simulink library "Body_Utilities"  (R2025a)
settings: Solver=VariableStepAuto  StartTime=0.0  StopTime=10.0  RelTol=1e-3
undefined symbols (not defined in the file or in its folder): Init, Vehicle, X, Y, Z
libraries: nesl_utility x38, sm_lib x9
Description:
  | Simscape Vehicle Templates Library
  | 
  | Copyright 2018-2026 The MathWorks, Inc.
settings Model: Creator=smiller  LastModifiedBy=smiller
settings OptimizationCC: ReuseModelBlockBuffer=off
settings ModelReferenceCC: EnableRefExpFcnMdlSchedulingChecks=on
settings RTWCC: GPUComputeCapability=3.5

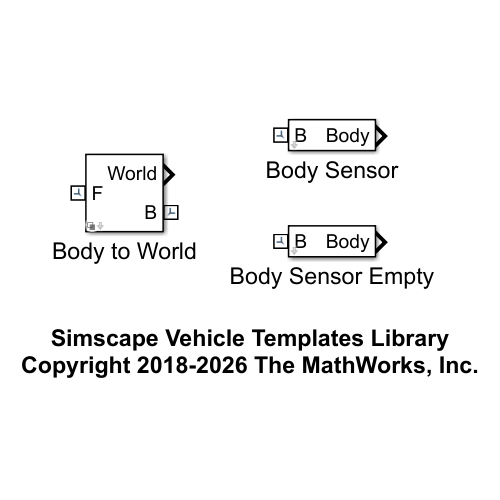
[thumbnail: Simulink's stored preview of the top-level diagram]
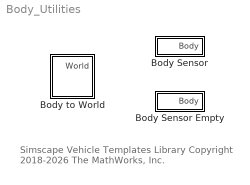
== system Body_Utilities ==
  note: Simscape Vehicle Templates Library
      | Copyright 2018-2026 The MathWorks, Inc.
  Body Sensor : Subsystem  mask{offset_body_sensor=Vehicle.Chassis.Body.sCG.Value}
      mask prompts: offset_body_sensor "Sensor Frame Offset [x y z] (m)"
  Body Sensor Empty : Subsystem  mask{offset_body_sensor=Vehicle.Chassis.Body.sCG.Value}
      mask prompts: offset_body_sensor "Sensor Frame Offset [x y z] (m)"
  Body to World : Subsystem  Variant=on  VariantControlMode=label  VariantControl=Choice  LabelModeActiveChoice=Free  mask{popup_BodyToWorld=Free, SpecifyPosTarget=on}
      mask prompts: popup_BodyToWorld "Body To World Connection"; SpecifyPosTarget "Specify Position Target"
      mask init:
      | bh = gcb;
      | b2w = get_param(bh,'popup_BodyToWorld');
      | set_param(bh,'LabelModeActiveChoice',b2w)
      | if(strcmp(b2w,'Free'))
      |     set_param([bh '/Free'],'SpecifyPosTarget',get_param(bh,'SpecifyPosTarget'));
      | end
      mask TypeOptions popup_BodyToWorld: Free | Rigid
      mask Display: disp(' ')

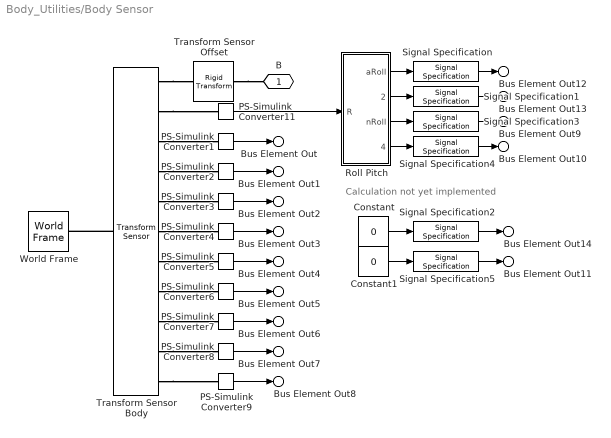
== system Body_Utilities/Body Sensor ==
  note: Calculation not yet implemented
  Constant : Constant  Value=0
  Constant1 : Constant  Value=0
  PS-Simulink Converter1 : nesl_utility/PS-Simulink Converter  PhysicalDomain=network_engine_domain  SubClassName=ps_output  LeftPortType=input  RightPortType=output  PseudoPeriodic=off  Frequencies=[]  VectorFormat=1-D array  Unit=m  AffineConversion=off
  PS-Simulink Converter11 : nesl_utility/PS-Simulink Converter  PhysicalDomain=network_engine_domain  SubClassName=ps_output  LeftPortType=input  RightPortType=output  PseudoPeriodic=off  Frequencies=[]  VectorFormat=1-D array  Unit=1  AffineConversion=off
  PS-Simulink Converter2 : nesl_utility/PS-Simulink Converter  PhysicalDomain=network_engine_domain  SubClassName=ps_output  LeftPortType=input  RightPortType=output  PseudoPeriodic=off  Frequencies=[]  VectorFormat=1-D array  Unit=m  AffineConversion=off
  PS-Simulink Converter3 : nesl_utility/PS-Simulink Converter  PhysicalDomain=network_engine_domain  SubClassName=ps_output  LeftPortType=input  RightPortType=output  PseudoPeriodic=off  Frequencies=[]  VectorFormat=1-D array  Unit=m  AffineConversion=off
  PS-Simulink Converter4 : nesl_utility/PS-Simulink Converter  PhysicalDomain=network_engine_domain  SubClassName=ps_output  LeftPortType=input  RightPortType=output  PseudoPeriodic=off  Frequencies=[]  VectorFormat=1-D array  Unit=m/s  AffineConversion=off
  PS-Simulink Converter5 : nesl_utility/PS-Simulink Converter  PhysicalDomain=network_engine_domain  SubClassName=ps_output  LeftPortType=input  RightPortType=output  PseudoPeriodic=off  Frequencies=[]  VectorFormat=1-D array  Unit=m/s  AffineConversion=off
  PS-Simulink Converter6 : nesl_utility/PS-Simulink Converter  PhysicalDomain=network_engine_domain  SubClassName=ps_output  LeftPortType=input  RightPortType=output  PseudoPeriodic=off  Frequencies=[]  VectorFormat=1-D array  Unit=m/s  AffineConversion=off
  PS-Simulink Converter7 : nesl_utility/PS-Simulink Converter  PhysicalDomain=network_engine_domain  SubClassName=ps_output  LeftPortType=input  RightPortType=output  PseudoPeriodic=off  Frequencies=[]  VectorFormat=1-D array  Unit=m/s^2  AffineConversion=off
  PS-Simulink Converter8 : nesl_utility/PS-Simulink Converter  PhysicalDomain=network_engine_domain  SubClassName=ps_output  LeftPortType=input  RightPortType=output  PseudoPeriodic=off  Frequencies=[]  VectorFormat=1-D array  Unit=m/s^2  AffineConversion=off
  PS-Simulink Converter9 : nesl_utility/PS-Simulink Converter  PhysicalDomain=network_engine_domain  SubClassName=ps_output  LeftPortType=input  RightPortType=output  PseudoPeriodic=off  Frequencies=[]  VectorFormat=1-D array  Unit=m/s^2  AffineConversion=off
  Roll Pitch : Subsystem
  Signal Specification : SignalSpecification  Unit=rad
  Signal Specification1 : SignalSpecification  Unit=rad
  Signal Specification2 : SignalSpecification  Unit=rad
  Signal Specification3 : SignalSpecification  Unit=rad/s
  Signal Specification4 : SignalSpecification  Unit=rad/s
  Signal Specification5 : SignalSpecification  Unit=rad/s
  Transform Sensor Offset : sm_lib/Frames and Transforms/Rigid Transform  RotationMethod=None  FollAlignAxisA=+X  BaseAlignAxisA=+Y  FollAlignAxisB=+Y  BaseAlignAxisB=+Z  RotationStandardAxis=+Z  RotationAngle=0.0  RotationAngleUnits=deg  RotationArbitraryAxis=[0 0 1]  RotationSequenceAxes=FollowerAxes  RotationSequence=XYX  RotationSequenceAngles=[0 0 0]  RotationSequenceAnglesUnits=deg  RotationMatrix=[1 0 0; 0 1 0; 0 0 1]  Quaternion=[1 0 0 0]  TranslationMethod=Cartesian  TranslationCartesianOffset=offset_body_sensor  TranslationCartesianOffsetUnits=m  TranslationStandardAxis=+Z  TranslationStandardOffset=0  TranslationStandardOffsetUnits=m  TranslationROffset=0  TranslationROffsetUnits=m  TranslationThetaOffset=0  TranslationThetaOffsetUnits=deg  TranslationZOffset=0  TranslationZOffsetUnits=m
  Transform Sensor Body : sm_lib/Frames and Transforms/Transform Sensor  MeasurementFrame=NonRotatingFollower  RotationSequence=XYX  SenseAngle=off  SenseAxis=off  SenseQ=off  SenseR=on  SenseRotationSequence=off  SenseOmegaX=off  SenseOmegaY=off  SenseOmegaZ=off  SenseOmega=off  SenseQDot=off  SenseRDot=off  SenseRotationSequenceDot=off  SenseAlphaX=off  SenseAlphaY=off  SenseAlphaZ=off  SenseAlpha=off  SenseQDDot=off  SenseRDDot=off  SenseX=on  SenseY=on  SenseZ=on  SenseXYZ=off  SenseRad=off  SenseAzim=off  SenseDist=off  SenseInc=off  SenseXDot=on  SenseYDot=on  SenseZDot=on  SenseXYZDot=off  SenseRadDot=off  SenseAzimDot=off  SenseDistDot=off  SenseIncDot=off  SenseXDDot=on  SenseYDDot=on  SenseZDDot=on  SenseXYZDDot=off  SenseRadDDot=off  SenseAzimDDot=off  SenseDistDDot=off  SenseIncDDot=off
  World Frame : sm_lib/Frames and Transforms/World Frame
  B : PMIOPort  Side=Left
  Bus Element Out : Outport  VectorParamsAs1DForOutWhenUnconnected=off  PortName=Body  Element=x
  Bus Element Out1 : Outport  VectorParamsAs1DForOutWhenUnconnected=off  PortName=Body  Element=y
  Bus Element Out2 : Outport  VectorParamsAs1DForOutWhenUnconnected=off  PortName=Body  Element=z
  Bus Element Out3 : Outport  VectorParamsAs1DForOutWhenUnconnected=off  PortName=Body  Element=vx
  Bus Element Out4 : Outport  VectorParamsAs1DForOutWhenUnconnected=off  PortName=Body  Element=vy
  Bus Element Out5 : Outport  VectorParamsAs1DForOutWhenUnconnected=off  PortName=Body  Element=vz
  Bus Element Out6 : Outport  VectorParamsAs1DForOutWhenUnconnected=off  PortName=Body  Element=gx
  Bus Element Out7 : Outport  VectorParamsAs1DForOutWhenUnconnected=off  PortName=Body  Element=gy
  Bus Element Out8 : Outport  VectorParamsAs1DForOutWhenUnconnected=off  PortName=Body  Element=gz
  Bus Element Out9 : Outport  VectorParamsAs1DForOutWhenUnconnected=off  PortName=Body  Element=nRoll
  Bus Element Out10 : Outport  VectorParamsAs1DForOutWhenUnconnected=off  PortName=Body  Element=nPitch
  Bus Element Out11 : Outport  VectorParamsAs1DForOutWhenUnconnected=off  PortName=Body  Element=nYaw
  Bus Element Out12 : Outport  VectorParamsAs1DForOutWhenUnconnected=off  PortName=Body  Element=aRoll
  Bus Element Out13 : Outport  VectorParamsAs1DForOutWhenUnconnected=off  PortName=Body  Element=aPitch
  Bus Element Out14 : Outport  VectorParamsAs1DForOutWhenUnconnected=off  PortName=Body  Element=aYaw
  wires:
  Roll Pitch/1(aRoll) -> Signal Specification/1
  Roll Pitch/2(aPitch) -> Signal Specification1/1
  Roll Pitch/4(nPitch) -> Signal Specification4/1
  Roll Pitch/3(nRoll) -> Signal Specification3/1
  Constant1/1 -> Signal Specification5/1
  Constant/1 -> Signal Specification2/1
  Signal Specification5/1 -> Bus Element Out11/1
  Signal Specification4/1 -> Bus Element Out10/1
  Signal Specification3/1 -> Bus Element Out9/1
  Signal Specification2/1 -> Bus Element Out14/1
  Signal Specification1/1 -> Bus Element Out13/1
  Signal Specification/1 -> Bus Element Out12/1
  PS-Simulink Converter4/1 -> Bus Element Out3/1
  PS-Simulink Converter1/1 -> Bus Element Out/1
  PS-Simulink Converter3/1 -> Bus Element Out2/1
  PS-Simulink Converter5/1 -> Bus Element Out4/1
  PS-Simulink Converter8/1 -> Bus Element Out7/1
  PS-Simulink Converter2/1 -> Bus Element Out1/1
  PS-Simulink Converter7/1 -> Bus Element Out6/1
  PS-Simulink Converter6/1 -> Bus Element Out5/1
  PS-Simulink Converter11/1 -> Roll Pitch/1(R)
  PS-Simulink Converter9/1 -> Bus Element Out8/1
  connections:
  Transform Sensor Body/RConn1 -- Transform Sensor Offset/RConn1
  Transform Sensor Body/RConn6 -- PS-Simulink Converter4/LConn1
  Transform Sensor Body/RConn8 -- PS-Simulink Converter6/LConn1
  Transform Sensor Body/RConn9 -- PS-Simulink Converter7/LConn1
  Transform Sensor Body/RConn10 -- PS-Simulink Converter8/LConn1
  Transform Sensor Offset/LConn1 -- B/RConn1
  Transform Sensor Body/LConn1 -- World Frame/RConn1
  Transform Sensor Body/RConn3 -- PS-Simulink Converter1/LConn1
  Transform Sensor Body/RConn7 -- PS-Simulink Converter5/LConn1
  Transform Sensor Body/RConn2 -- PS-Simulink Converter11/LConn1
  Transform Sensor Body/RConn11 -- PS-Simulink Converter9/LConn1
  Transform Sensor Body/RConn4 -- PS-Simulink Converter2/LConn1
  Transform Sensor Body/RConn5 -- PS-Simulink Converter3/LConn1

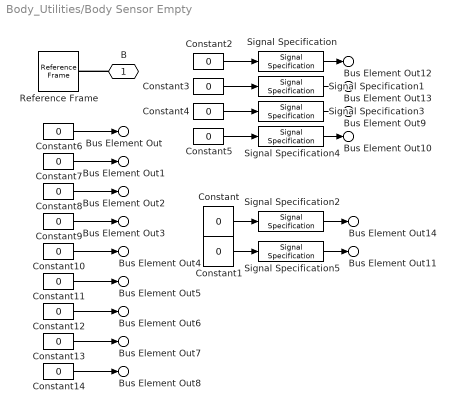
== system Body_Utilities/Body Sensor Empty ==
  Constant{,1..14} (15 alike) : Constant  Value=0
  Reference Frame : sm_lib/Frames and Transforms/Reference Frame
  Signal Specification : SignalSpecification  Unit=rad
  Signal Specification1 : SignalSpecification  Unit=rad
  Signal Specification2 : SignalSpecification  Unit=rad
  Signal Specification3 : SignalSpecification  Unit=rad/s
  Signal Specification4 : SignalSpecification  Unit=rad/s
  Signal Specification5 : SignalSpecification  Unit=rad/s
  B : PMIOPort  Side=Left
  Bus Element Out : Outport  VectorParamsAs1DForOutWhenUnconnected=off  PortName=Body  Element=x
  Bus Element Out1 : Outport  VectorParamsAs1DForOutWhenUnconnected=off  PortName=Body  Element=y
  Bus Element Out2 : Outport  VectorParamsAs1DForOutWhenUnconnected=off  PortName=Body  Element=z
  Bus Element Out3 : Outport  VectorParamsAs1DForOutWhenUnconnected=off  PortName=Body  Element=vx
  Bus Element Out4 : Outport  VectorParamsAs1DForOutWhenUnconnected=off  PortName=Body  Element=vy
  Bus Element Out5 : Outport  VectorParamsAs1DForOutWhenUnconnected=off  PortName=Body  Element=vz
  Bus Element Out6 : Outport  VectorParamsAs1DForOutWhenUnconnected=off  PortName=Body  Element=gx
  Bus Element Out7 : Outport  VectorParamsAs1DForOutWhenUnconnected=off  PortName=Body  Element=gy
  Bus Element Out8 : Outport  VectorParamsAs1DForOutWhenUnconnected=off  PortName=Body  Element=gz
  Bus Element Out9 : Outport  VectorParamsAs1DForOutWhenUnconnected=off  PortName=Body  Element=nRoll
  Bus Element Out10 : Outport  VectorParamsAs1DForOutWhenUnconnected=off  PortName=Body  Element=nPitch
  Bus Element Out11 : Outport  VectorParamsAs1DForOutWhenUnconnected=off  PortName=Body  Element=nYaw
  Bus Element Out12 : Outport  VectorParamsAs1DForOutWhenUnconnected=off  PortName=Body  Element=aRoll
  Bus Element Out13 : Outport  VectorParamsAs1DForOutWhenUnconnected=off  PortName=Body  Element=aPitch
  Bus Element Out14 : Outport  VectorParamsAs1DForOutWhenUnconnected=off  PortName=Body  Element=aYaw
  wires:
  Constant14/1 -> Bus Element Out8/1
  Constant11/1 -> Bus Element Out5/1
  Constant12/1 -> Bus Element Out6/1
  Constant7/1 -> Bus Element Out1/1
  Constant13/1 -> Bus Element Out7/1
  Constant10/1 -> Bus Element Out4/1
  Constant8/1 -> Bus Element Out2/1
  Constant6/1 -> Bus Element Out/1
  Constant9/1 -> Bus Element Out3/1
  Signal Specification/1 -> Bus Element Out12/1
  Signal Specification1/1 -> Bus Element Out13/1
  Signal Specification2/1 -> Bus Element Out14/1
  Signal Specification3/1 -> Bus Element Out9/1
  Signal Specification4/1 -> Bus Element Out10/1
  Signal Specification5/1 -> Bus Element Out11/1
  Constant/1 -> Signal Specification2/1
  Constant1/1 -> Signal Specification5/1
  Constant4/1 -> Signal Specification3/1
  Constant5/1 -> Signal Specification4/1
  Constant3/1 -> Signal Specification1/1
  Constant2/1 -> Signal Specification/1
  connections:
  B/RConn1 -- Reference Frame/RConn1

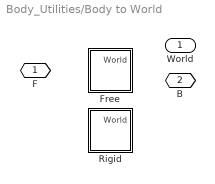
== system Body_Utilities/Body to World ==
  Free : Subsystem  VariantControl=Free  mask(Body to World){Init=Init.Chassis, SpecifyPosTarget=on}
      mask prompts: Init "Initial Values"; SpecifyPosTarget "Specify Position Target"
      mask help: Models the connection between the vehicle body and world. Permits 6 degrees of freedom and sets the initial position, orientation, and speed of the vehicle body.
      mask init:
      | initial_aveh = [Init.aChassis.Value(3) Init.aChassis.Value(2) Init.aChassis.Value(1)];
      | rotmat_ypr = sm_car_yawpitchroll_to_rotmat(Init.aChassis.Value(3),Init.aChassis.Value(2),Init.aChassis.Value(1));
      | initial_vveh = rotmat_ypr*(Init.vChassis.Value)';
      | 
      | sptState = get_param(gcb,'SpecifyPosTarget');
      | 
      | set_param([gcb '/Body World Joint'],...
      |         'PxPositionTargetSpecify',sptState,...
      |         'PyPositionTargetSpecify',sptState,...
      |         'PzPositionTargetSpecify',sptState,...
      |         'SphPositionTargetSpecify',sptState,...
      |         'PxVelocityTargetSpecify',sptState,...
      |         'PyVelocityTargetSpecify',sptState,...
      |         'PzVelocityTargetSpecify',sptState,...
      |         'SphVelocityTargetSpecify',sptState...
      |         );
      mask Help: web('sm_car_doc_body_to_world.html')
  Rigid : Subsystem  VariantControl=Rigid  mask(Body to World){Init=Init.Chassis}
      mask prompts: Init "Initial Values"
      mask help: Models the connection between the vehicle body and world. Permits 6 degrees of freedom and sets the initial position, orientation, and speed of the vehicle body.
      mask init:
      | initial_aveh = [Init.aChassis.Value(3) Init.aChassis.Value(2) Init.aChassis.Value(1)];
      | rotmat_ypr = sm_car_yawpitchroll_to_rotmat(Init.aChassis.Value(3),Init.aChassis.Value(2),Init.aChassis.Value(1));
      | initial_vveh = rotmat_ypr*(Init.vChassis.Value)';
      mask Help: web('sm_car_doc_body_to_world.html')
  F : PMIOPort  Side=Left
  B : PMIOPort  Port=2  Side=Right
  World : Outport

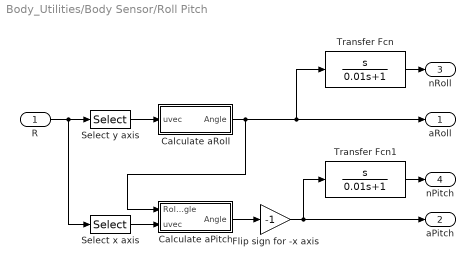
== system Body_Utilities/Body Sensor/Roll Pitch ==
  R : Inport
  Calculate aPitch : Subsystem
  Calculate aRoll : Subsystem
  "Flip sign for -x axis " : Gain  Gain=-1
  Select x axis : Selector  NumberOfDimensions=2  InputPortWidth=2  IndexOptions=Index vector (dialog),Index vector (dialog)  Indices=[1 2 3],1  OutputSizes=1,1
  Select y axis : Selector  NumberOfDimensions=2  InputPortWidth=2  IndexOptions=Index vector (dialog),Index vector (dialog)  Indices=[1 2 3],2  OutputSizes=1,1
  Transfer Fcn : TransferFcn  Numerator=[1 0]  Denominator=[0.01 1]
  Transfer Fcn1 : TransferFcn  Numerator=[1 0]  Denominator=[0.01 1]
  aRoll : Outport  VectorParamsAs1DForOutWhenUnconnected=off
  aPitch : Outport  Port=2  VectorParamsAs1DForOutWhenUnconnected=off
  nRoll : Outport  Port=3  VectorParamsAs1DForOutWhenUnconnected=off
  nPitch : Outport  Port=4  VectorParamsAs1DForOutWhenUnconnected=off
  wires:
  Transfer Fcn1/1 -> nPitch/1
  Transfer Fcn/1 -> nRoll/1
  Calculate aRoll/1(Angle) -> Calculate aPitch/1(Roll Angle), aRoll/1, Transfer Fcn/1
  "Flip sign for -x axis "/1 -> Transfer Fcn1/1, aPitch/1
  Select y axis/1 -> Calculate aRoll/1(uvec)
  R/1 -> Select x axis/1, Select y axis/1
  Select x axis/1 -> Calculate aPitch/2(uvec)
  Calculate aPitch/1(Angle) -> "Flip sign for -x axis "/1

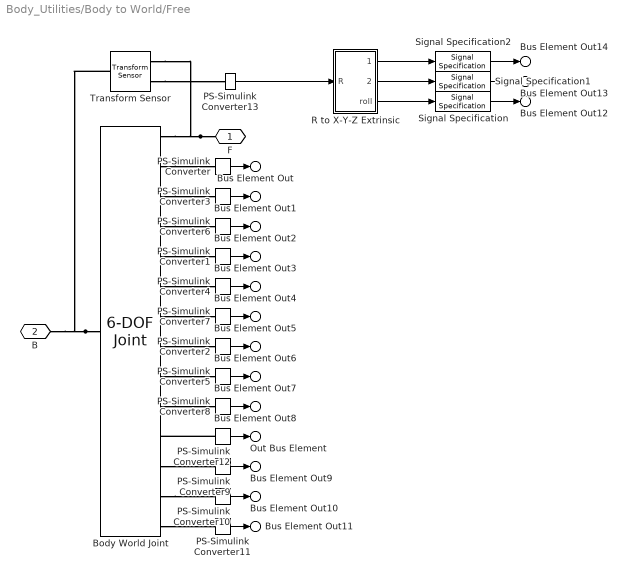
== system Body_Utilities/Body to World/Free ==
  Body World Joint : sm_lib/Joints/6-DOF Joint  JointMode=Normal  CompositeWrenchDir=FollowerOnBase  CompositeWrenchFrame=BaseFrame  SenseConstraintForce=off  SenseConstraintTorque=off  SenseTotalForce=off  SenseTotalTorque=off  PxPositionTargetSpecify=on  PxPositionTargetPriority=Low  PxPositionTargetValue=Init.sChassis.Value(1)  PxPositionTargetValueUnits=m  PxVelocityTargetSpecify=on  PxVelocityTargetPriority=Low  PxVelocityTargetValue=initial_vveh(1)  PxVelocityTargetValueUnits=m/s  PxEquilibriumPosition=0  PxEquilibriumPositionUnits=m  PxSpringStiffness=0  PxSpringStiffnessUnits=N/m  PxDampingCoefficient=0  PxDampingCoefficientUnits=N/(m/s)  PxLowerLimitSpecify=off  PxLowerLimitBound=-1  PxLowerLimitBoundUnits=m  PxLowerLimitStiffness=1e6  PxLowerLimitStiffnessUnits=N/m  PxLowerLimitDamping=1e3  PxLowerLimitDampingUnits=N/(m/s)  PxLowerLimitTransitionRegionWidth=1e-4  PxLowerLimitTransitionRegionWidthUnits=m  PxUpperLimitSpecify=off  PxUpperLimitBound=1  PxUpperLimitBoundUnits=m  PxUpperLimitStiffness=1e6  PxUpperLimitStiffnessUnits=N/m  PxUpperLimitDamping=1e3  PxUpperLimitDampingUnits=N/(m/s)  PxUpperLimitTransitionRegionWidth=1e-4  PxUpperLimitTransitionRegionWidthUnits=m  PxTorqueActuationMode=NoTorque  PxMotionActuationMode=ComputedMotion  PxSensePosition=on  PxSenseVelocity=on  PxSenseAcceleration=on  PxSenseTorqueForce=off  PxSenseLowerLimitTorqueForce=off  PxSenseUpperLimitTorqueForce=off  PyPositionTargetSpecify=on  PyPositionTargetPriority=Low  PyPositionTargetValue=Init.sChassis.Value(2)  PyPositionTargetValueUnits=m  PyVelocityTargetSpecify=on  PyVelocityTargetPriority=Low  PyVelocityTargetValue=initial_vveh(2)  PyVelocityTargetValueUnits=m/s  PyEquilibriumPosition=0  PyEquilibriumPositionUnits=m  PySpringStiffness=0  PySpringStiffnessUnits=N/m  PyDampingCoefficient=0  PyDampingCoefficientUnits=N/(m/s)  PyLowerLimitSpecify=off  PyLowerLimitBound=-1  PyLowerLimitBoundUnits=m  PyLowerLimitStiffness=1e6  PyLowerLimitStiffnessUnits=N/m  PyLowerLimitDamping=1e3  PyLowerLimitDampingUnits=N/(m/s)  PyLowerLimitTransitionRegionWidth=1e-4  PyLowerLimitTransitionRegionWidthUnits=m  PyUpperLimitSpecify=off  PyUpperLimitBound=1  PyUpperLimitBoundUnits=m  PyUpperLimitStiffness=1e6  PyUpperLimitStiffnessUnits=N/m  PyUpperLimitDamping=1e3  PyUpperLimitDampingUnits=N/(m/s)  PyUpperLimitTransitionRegionWidth=1e-4  PyUpperLimitTransitionRegionWidthUnits=m  PyTorqueActuationMode=NoTorque  PyMotionActuationMode=ComputedMotion  PySensePosition=on  PySenseVelocity=on  PySenseAcceleration=on  PySenseTorqueForce=off  PySenseLowerLimitTorqueForce=off  PySenseUpperLimitTorqueForce=off  PzPositionTargetSpecify=on  PzPositionTargetPriority=Low  PzPositionTargetValue=Init.sChassis.Value(3)  PzPositionTargetValueUnits=m  PzVelocityTargetSpecify=on  PzVelocityTargetPriority=Low  PzVelocityTargetValue=initial_vveh(3)  PzVelocityTargetValueUnits=m/s  PzEquilibriumPosition=0  PzEquilibriumPositionUnits=m  PzSpringStiffness=0  PzSpringStiffnessUnits=N/m  PzDampingCoefficient=0  PzDampingCoefficientUnits=N/(m/s)  PzLowerLimitSpecify=off  PzLowerLimitBound=-1  PzLowerLimitBoundUnits=m  PzLowerLimitStiffness=1e6  PzLowerLimitStiffnessUnits=N/m  PzLowerLimitDamping=1e3  PzLowerLimitDampingUnits=N/(m/s)  PzLowerLimitTransitionRegionWidth=1e-4  PzLowerLimitTransitionRegionWidthUnits=m  PzUpperLimitSpecify=off  PzUpperLimitBound=1  PzUpperLimitBoundUnits=m  PzUpperLimitStiffness=1e6  PzUpperLimitStiffnessUnits=N/m  PzUpperLimitDamping=1e3  PzUpperLimitDampingUnits=N/(m/s)  PzUpperLimitTransitionRegionWidth=1e-4  PzUpperLimitTransitionRegionWidthUnits=m  PzTorqueActuationMode=NoTorque  PzMotionActuationMode=ComputedMotion  PzSensePosition=on  PzSenseVelocity=on  PzSenseAcceleration=on  PzSenseTorqueForce=off  PzSenseLowerLimitTorqueForce=off  PzSenseUpperLimitTorqueForce=off  SphPositionTargetSpecify=on  SphPositionTargetPriority=Low  SphPositionTargetRotationMethod=RotationSequence  SphPositionTargetFollAlignAxisA=+X  SphPositionTargetBaseAlignAxisA=+Y  SphPositionTargetFollAlignAxisB=+Y  SphPositionTargetBaseAlignAxisB=+Z  SphPositionTargetRotationStandardAxis=+Z  SphPositionTargetRotationAngle=0.0  SphPositionTargetRotationAngleUnits=deg  SphPositionTargetRotationArbitraryAxis=[0 0 1]  SphPositionTargetRotationSequenceAxes=FollowerAxes  SphPositionTargetRotationSequence=ZYX  SphPositionTargetRotationSequenceAngles=initial_aveh  SphPositionTargetRotationSequenceAnglesUnits=rad  SphPositionTargetRotationMatrix=[1 0 0; 0 1 0; 0 0 1]  SphPositionTargetQuaternion=[1 0 0 0]  SphVelocityTargetSpecify=on  SphVelocityTargetPriority=Low  SphVelocityTargetValue=[0 0 0]  SphVelocityTargetValueUnits=deg/s  SphVelocityTargetInFollowerFrame=on  SphEqPosRotationMethod=None  SphEqPosFollAlignAxisA=+X  SphEqPosBaseAlignAxisA=+Y  SphEqPosFollAlignAxisB=+Y  SphEqPosBaseAlignAxisB=+Z  SphEqPosRotationStandardAxis=+Z  SphEqPosRotationAngle=0.0  SphEqPosRotationAngleUnits=deg  SphEqPosRotationArbitraryAxis=[0 0 1]  SphEqPosRotationSequenceAxes=FollowerAxes  SphEqPosRotationSequence=XYX  SphEqPosRotationSequenceAngles=[0 0 0]  SphEqPosRotationSequenceAnglesUnits=deg  SphEqPosRotationMatrix=[1 0 0; 0 1 0; 0 0 1]  SphEqPosQuaternion=[1 0 0 0]  SphSpringStiffness=0  SphSpringStiffnessUnits=N*m/deg  SphDampingCoefficient=0  SphDampingCoefficientUnits=N*m/(deg/s)  SphLowerLimitSpecify=off  SphLowerLimitBound=15  SphLowerLimitBoundUnits=deg  SphLowerLimitStiffness=1e4  SphLowerLimitStiffnessUnits=N*m/deg  SphLowerLimitDamping=10  SphLowerLimitDampingUnits=N*m/(deg/s)  SphLowerLimitTransitionRegionWidth=0.1  SphLowerLimitTransitionRegionWidthUnits=deg  SphUpperLimitSpecify=off  SphUpperLimitBound=45  SphUpperLimitBoundUnits=deg  SphUpperLimitStiffness=1e4  SphUpperLimitStiffnessUnits=N*m/deg  SphUpperLimitDamping=10  SphUpperLimitDampingUnits=N*m/(deg/s)  SphUpperLimitTransitionRegionWidth=0.1  SphUpperLimitTransitionRegionWidthUnits=deg  SphTorqueActuationMode=NoTorque  SphActuateTorqueX=off  SphActuateTorqueY=off  SphActuateTorqueZ=off  SphActuateTorque=off  SphActuationFrame=BaseFrame  SphSensePosition=on  SphSenseVelocityX=on  SphSenseVelocityY=on  SphSenseVelocityZ=on  SphSenseVelocity=off  SphSenseAccelerationX=off  SphSenseAccelerationY=off  SphSenseAccelerationZ=off  SphSenseAcceleration=off  SphSenseLowerLimitTorqueMag=off  SphSenseUpperLimitTorqueMag=off  SphSensingFrame=BaseFrame
  PS-Simulink Converter : nesl_utility/PS-Simulink Converter  PhysicalDomain=network_engine_domain  SubClassName=ps_output  LeftPortType=input  RightPortType=output  PseudoPeriodic=off  Frequencies=[]  VectorFormat=1-D array  Unit=m  AffineConversion=off
  PS-Simulink Converter1 : nesl_utility/PS-Simulink Converter  PhysicalDomain=network_engine_domain  SubClassName=ps_output  LeftPortType=input  RightPortType=output  PseudoPeriodic=off  Frequencies=[]  VectorFormat=1-D array  Unit=m  AffineConversion=off
  PS-Simulink Converter10 : nesl_utility/PS-Simulink Converter  PhysicalDomain=network_engine_domain  SubClassName=ps_output  LeftPortType=input  RightPortType=output  PseudoPeriodic=off  Frequencies=[]  VectorFormat=1-D array  Unit=rad/s  AffineConversion=off
  PS-Simulink Converter11 : nesl_utility/PS-Simulink Converter  PhysicalDomain=network_engine_domain  SubClassName=ps_output  LeftPortType=input  RightPortType=output  PseudoPeriodic=off  Frequencies=[]  VectorFormat=1-D array  Unit=rad/s  AffineConversion=off
  PS-Simulink Converter12 : nesl_utility/PS-Simulink Converter  PhysicalDomain=network_engine_domain  SubClassName=ps_output  LeftPortType=input  RightPortType=output  PseudoPeriodic=off  Frequencies=[]  VectorFormat=1-D array  Unit=1  AffineConversion=off
  PS-Simulink Converter13 : nesl_utility/PS-Simulink Converter  PhysicalDomain=network_engine_domain  SubClassName=ps_output  LeftPortType=input  RightPortType=output  PseudoPeriodic=off  Frequencies=[]  VectorFormat=1-D array  Unit=1  AffineConversion=off
  PS-Simulink Converter2 : nesl_utility/PS-Simulink Converter  PhysicalDomain=network_engine_domain  SubClassName=ps_output  LeftPortType=input  RightPortType=output  PseudoPeriodic=off  Frequencies=[]  VectorFormat=1-D array  Unit=m  AffineConversion=off
  PS-Simulink Converter3 : nesl_utility/PS-Simulink Converter  PhysicalDomain=network_engine_domain  SubClassName=ps_output  LeftPortType=input  RightPortType=output  PseudoPeriodic=off  Frequencies=[]  VectorFormat=1-D array  Unit=m/s  AffineConversion=off
  PS-Simulink Converter4 : nesl_utility/PS-Simulink Converter  PhysicalDomain=network_engine_domain  SubClassName=ps_output  LeftPortType=input  RightPortType=output  PseudoPeriodic=off  Frequencies=[]  VectorFormat=1-D array  Unit=m/s  AffineConversion=off
  PS-Simulink Converter5 : nesl_utility/PS-Simulink Converter  PhysicalDomain=network_engine_domain  SubClassName=ps_output  LeftPortType=input  RightPortType=output  PseudoPeriodic=off  Frequencies=[]  VectorFormat=1-D array  Unit=m/s  AffineConversion=off
  PS-Simulink Converter6 : nesl_utility/PS-Simulink Converter  PhysicalDomain=network_engine_domain  SubClassName=ps_output  LeftPortType=input  RightPortType=output  PseudoPeriodic=off  Frequencies=[]  VectorFormat=1-D array  Unit=m/s^2  AffineConversion=off
  PS-Simulink Converter7 : nesl_utility/PS-Simulink Converter  PhysicalDomain=network_engine_domain  SubClassName=ps_output  LeftPortType=input  RightPortType=output  PseudoPeriodic=off  Frequencies=[]  VectorFormat=1-D array  Unit=m/s^2  AffineConversion=off
  PS-Simulink Converter8 : nesl_utility/PS-Simulink Converter  PhysicalDomain=network_engine_domain  SubClassName=ps_output  LeftPortType=input  RightPortType=output  PseudoPeriodic=off  Frequencies=[]  VectorFormat=1-D array  Unit=m/s^2  AffineConversion=off
  PS-Simulink Converter9 : nesl_utility/PS-Simulink Converter  PhysicalDomain=network_engine_domain  SubClassName=ps_output  LeftPortType=input  RightPortType=output  PseudoPeriodic=off  Frequencies=[]  VectorFormat=1-D array  Unit=rad/s  AffineConversion=off
  R to X-Y-Z Extrinsic : Subsystem  mask(Rotation Matrix to X-Y-Z Extrinsic){}
      mask help: Computes roll / pitch / yaw values assuming they correspond to X, Y, and Z rotations, applied in that order and using extrinsic rotations (rotations applied about the fixed axes of the base frame). Does not handle case where Y (pitch) rotation is +/-90 degrees.
  Signal Specification : SignalSpecification  Unit=rad
  Signal Specification1 : SignalSpecification  Unit=rad
  Signal Specification2 : SignalSpecification  Unit=rad
  Transform Sensor : sm_lib/Frames and Transforms/Transform Sensor  MeasurementFrame=World  RotationSequence=XYX  SenseAngle=off  SenseAxis=off  SenseQ=off  SenseR=on  SenseRotationSequence=off  SenseOmegaX=off  SenseOmegaY=off  SenseOmegaZ=off  SenseOmega=off  SenseQDot=off  SenseRDot=off  SenseRotationSequenceDot=off  SenseAlphaX=off  SenseAlphaY=off  SenseAlphaZ=off  SenseAlpha=off  SenseQDDot=off  SenseRDDot=off  SenseX=off  SenseY=off  SenseZ=off  SenseXYZ=off  SenseRad=off  SenseAzim=off  SenseDist=off  SenseInc=off  SenseXDot=off  SenseYDot=off  SenseZDot=off  SenseXYZDot=off  SenseRadDot=off  SenseAzimDot=off  SenseDistDot=off  SenseIncDot=off  SenseXDDot=off  SenseYDDot=off  SenseZDDot=off  SenseXYZDDot=off  SenseRadDDot=off  SenseAzimDDot=off  SenseDistDDot=off  SenseIncDDot=off
  F : PMIOPort  Side=Left
  B : PMIOPort  Port=2  Side=Right
  Bus Element Out : Outport  VectorParamsAs1DForOutWhenUnconnected=off  PortName=World  Element=x
  Bus Element Out3 : Outport  VectorParamsAs1DForOutWhenUnconnected=off  PortName=World  Element=y
  Bus Element Out6 : Outport  VectorParamsAs1DForOutWhenUnconnected=off  PortName=World  Element=z
  Bus Element Out1 : Outport  VectorParamsAs1DForOutWhenUnconnected=off  PortName=World  Element=vx
  Bus Element Out4 : Outport  VectorParamsAs1DForOutWhenUnconnected=off  PortName=World  Element=vy
  Bus Element Out7 : Outport  VectorParamsAs1DForOutWhenUnconnected=off  PortName=World  Element=vz
  Bus Element Out2 : Outport  VectorParamsAs1DForOutWhenUnconnected=off  PortName=World  Element=gx
  Bus Element Out5 : Outport  VectorParamsAs1DForOutWhenUnconnected=off  PortName=World  Element=gy
  Bus Element Out8 : Outport  VectorParamsAs1DForOutWhenUnconnected=off  PortName=World  Element=gz
  Bus Element Out9 : Outport  VectorParamsAs1DForOutWhenUnconnected=off  PortName=World  Element=nRoll
  Bus Element Out10 : Outport  VectorParamsAs1DForOutWhenUnconnected=off  PortName=World  Element=nPitch
  Bus Element Out11 : Outport  VectorParamsAs1DForOutWhenUnconnected=off  PortName=World  Element=nYaw
  Bus Element Out12 : Outport  VectorParamsAs1DForOutWhenUnconnected=off  PortName=World  Element=aRoll
  Bus Element Out13 : Outport  VectorParamsAs1DForOutWhenUnconnected=off  PortName=World  Element=aPitch
  Bus Element Out14 : Outport  VectorParamsAs1DForOutWhenUnconnected=off  PortName=World  Element=aYaw
  Out Bus Element : Outport  VectorParamsAs1DForOutWhenUnconnected=off  PortName=World  Element=Q
  wires:
  R to X-Y-Z Extrinsic/1(yaw) -> Signal Specification2/1
  R to X-Y-Z Extrinsic/3(roll) -> Signal Specification/1
  R to X-Y-Z Extrinsic/2(pitch) -> Signal Specification1/1
  PS-Simulink Converter13/1 -> R to X-Y-Z Extrinsic/1(R)
  PS-Simulink Converter12/1 -> Out Bus Element/1
  PS-Simulink Converter11/1 -> Bus Element Out11/1
  PS-Simulink Converter10/1 -> Bus Element Out10/1
  Signal Specification/1 -> Bus Element Out12/1
  Signal Specification1/1 -> Bus Element Out13/1
  Signal Specification2/1 -> Bus Element Out14/1
  PS-Simulink Converter3/1 -> Bus Element Out1/1
  PS-Simulink Converter2/1 -> Bus Element Out6/1
  PS-Simulink Converter6/1 -> Bus Element Out2/1
  PS-Simulink Converter4/1 -> Bus Element Out4/1
  PS-Simulink Converter/1 -> Bus Element Out/1
  PS-Simulink Converter5/1 -> Bus Element Out7/1
  PS-Simulink Converter9/1 -> Bus Element Out9/1
  PS-Simulink Converter8/1 -> Bus Element Out8/1
  PS-Simulink Converter7/1 -> Bus Element Out5/1
  PS-Simulink Converter1/1 -> Bus Element Out3/1
  connections:
  Transform Sensor/RConn2 -- PS-Simulink Converter13/LConn1
  PS-Simulink Converter12/LConn1 -- Body World Joint/RConn11
  Body World Joint/RConn8 -- PS-Simulink Converter2/LConn1
  Body World Joint/RConn9 -- PS-Simulink Converter5/LConn1
  F/RConn1 -- Transform Sensor/RConn1 -- Body World Joint/RConn1
  Body World Joint/RConn3 -- PS-Simulink Converter3/LConn1
  Body World Joint/RConn10 -- PS-Simulink Converter8/LConn1
  Body World Joint/RConn4 -- PS-Simulink Converter6/LConn1
  Body World Joint/RConn2 -- PS-Simulink Converter/LConn1
  Body World Joint/RConn7 -- PS-Simulink Converter7/LConn1
  Body World Joint/RConn13 -- PS-Simulink Converter10/LConn1
  Body World Joint/RConn14 -- PS-Simulink Converter11/LConn1
  Body World Joint/RConn5 -- PS-Simulink Converter1/LConn1
  Body World Joint/LConn1 -- Transform Sensor/LConn1 -- B/RConn1
  Body World Joint/RConn12 -- PS-Simulink Converter9/LConn1
  Body World Joint/RConn6 -- PS-Simulink Converter4/LConn1

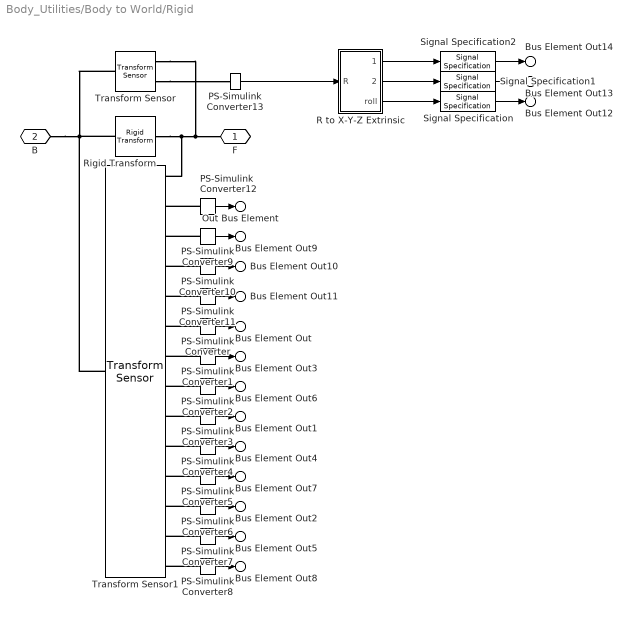
== system Body_Utilities/Body to World/Rigid ==
  PS-Simulink Converter : nesl_utility/PS-Simulink Converter  PhysicalDomain=network_engine_domain  SubClassName=ps_output  LeftPortType=input  RightPortType=output  PseudoPeriodic=off  Frequencies=[]  VectorFormat=1-D array  Unit=m  AffineConversion=off
  PS-Simulink Converter1 : nesl_utility/PS-Simulink Converter  PhysicalDomain=network_engine_domain  SubClassName=ps_output  LeftPortType=input  RightPortType=output  PseudoPeriodic=off  Frequencies=[]  VectorFormat=1-D array  Unit=m  AffineConversion=off
  PS-Simulink Converter10 : nesl_utility/PS-Simulink Converter  PhysicalDomain=network_engine_domain  SubClassName=ps_output  LeftPortType=input  RightPortType=output  PseudoPeriodic=off  Frequencies=[]  VectorFormat=1-D array  Unit=rad/s  AffineConversion=off
  PS-Simulink Converter11 : nesl_utility/PS-Simulink Converter  PhysicalDomain=network_engine_domain  SubClassName=ps_output  LeftPortType=input  RightPortType=output  PseudoPeriodic=off  Frequencies=[]  VectorFormat=1-D array  Unit=rad/s  AffineConversion=off
  PS-Simulink Converter12 : nesl_utility/PS-Simulink Converter  PhysicalDomain=network_engine_domain  SubClassName=ps_output  LeftPortType=input  RightPortType=output  PseudoPeriodic=off  Frequencies=[]  VectorFormat=1-D array  Unit=1  AffineConversion=off
  PS-Simulink Converter13 : nesl_utility/PS-Simulink Converter  PhysicalDomain=network_engine_domain  SubClassName=ps_output  LeftPortType=input  RightPortType=output  PseudoPeriodic=off  Frequencies=[]  VectorFormat=1-D array  Unit=1  AffineConversion=off
  PS-Simulink Converter2 : nesl_utility/PS-Simulink Converter  PhysicalDomain=network_engine_domain  SubClassName=ps_output  LeftPortType=input  RightPortType=output  PseudoPeriodic=off  Frequencies=[]  VectorFormat=1-D array  Unit=m  AffineConversion=off
  PS-Simulink Converter3 : nesl_utility/PS-Simulink Converter  PhysicalDomain=network_engine_domain  SubClassName=ps_output  LeftPortType=input  RightPortType=output  PseudoPeriodic=off  Frequencies=[]  VectorFormat=1-D array  Unit=m/s  AffineConversion=off
  PS-Simulink Converter4 : nesl_utility/PS-Simulink Converter  PhysicalDomain=network_engine_domain  SubClassName=ps_output  LeftPortType=input  RightPortType=output  PseudoPeriodic=off  Frequencies=[]  VectorFormat=1-D array  Unit=m/s  AffineConversion=off
  PS-Simulink Converter5 : nesl_utility/PS-Simulink Converter  PhysicalDomain=network_engine_domain  SubClassName=ps_output  LeftPortType=input  RightPortType=output  PseudoPeriodic=off  Frequencies=[]  VectorFormat=1-D array  Unit=m/s  AffineConversion=off
  PS-Simulink Converter6 : nesl_utility/PS-Simulink Converter  PhysicalDomain=network_engine_domain  SubClassName=ps_output  LeftPortType=input  RightPortType=output  PseudoPeriodic=off  Frequencies=[]  VectorFormat=1-D array  Unit=m/s^2  AffineConversion=off
  PS-Simulink Converter7 : nesl_utility/PS-Simulink Converter  PhysicalDomain=network_engine_domain  SubClassName=ps_output  LeftPortType=input  RightPortType=output  PseudoPeriodic=off  Frequencies=[]  VectorFormat=1-D array  Unit=m/s^2  AffineConversion=off
  PS-Simulink Converter8 : nesl_utility/PS-Simulink Converter  PhysicalDomain=network_engine_domain  SubClassName=ps_output  LeftPortType=input  RightPortType=output  PseudoPeriodic=off  Frequencies=[]  VectorFormat=1-D array  Unit=m/s^2  AffineConversion=off
  PS-Simulink Converter9 : nesl_utility/PS-Simulink Converter  PhysicalDomain=network_engine_domain  SubClassName=ps_output  LeftPortType=input  RightPortType=output  PseudoPeriodic=off  Frequencies=[]  VectorFormat=1-D array  Unit=rad/s  AffineConversion=off
  R to X-Y-Z Extrinsic : Subsystem  mask(Rotation Matrix to X-Y-Z Extrinsic){}
      mask help: Computes roll / pitch / yaw values assuming they correspond to X, Y, and Z rotations, applied in that order and using extrinsic rotations (rotations applied about the fixed axes of the base frame). Does not handle case where Y (pitch) rotation is +/-90 degrees.
  Rigid Transform : sm_lib/Frames and Transforms/Rigid Transform  RotationMethod=RotationSequence  FollAlignAxisA=+X  BaseAlignAxisA=+Y  FollAlignAxisB=+Y  BaseAlignAxisB=+Z  RotationStandardAxis=+Z  RotationAngle=0.0  RotationAngleUnits=deg  RotationArbitraryAxis=[0 0 1]  RotationSequenceAxes=FollowerAxes  RotationSequence=ZYX  RotationSequenceAngles=initial_aveh  RotationSequenceAnglesUnits=rad  RotationMatrix=[1 0 0; 0 1 0; 0 0 1]  Quaternion=[1 0 0 0]  TranslationMethod=Cartesian  TranslationCartesianOffset=[Init.sChassis.Value(1) Init.sChassis.Value(2) Init.sChassis.Value(3)]  TranslationCartesianOffsetUnits=m  TranslationStandardAxis=+Z  TranslationStandardOffset=0  TranslationStandardOffsetUnits=m  TranslationROffset=0  TranslationROffsetUnits=m  TranslationThetaOffset=0  TranslationThetaOffsetUnits=deg  TranslationZOffset=0  TranslationZOffsetUnits=m
  Signal Specification : SignalSpecification  Unit=rad
  Signal Specification1 : SignalSpecification  Unit=rad
  Signal Specification2 : SignalSpecification  Unit=rad
  Transform Sensor : sm_lib/Frames and Transforms/Transform Sensor  MeasurementFrame=World  RotationSequence=XYX  SenseAngle=off  SenseAxis=off  SenseQ=off  SenseR=on  SenseRotationSequence=off  SenseOmegaX=off  SenseOmegaY=off  SenseOmegaZ=off  SenseOmega=off  SenseQDot=off  SenseRDot=off  SenseRotationSequenceDot=off  SenseAlphaX=off  SenseAlphaY=off  SenseAlphaZ=off  SenseAlpha=off  SenseQDDot=off  SenseRDDot=off  SenseX=off  SenseY=off  SenseZ=off  SenseXYZ=off  SenseRad=off  SenseAzim=off  SenseDist=off  SenseInc=off  SenseXDot=off  SenseYDot=off  SenseZDot=off  SenseXYZDot=off  SenseRadDot=off  SenseAzimDot=off  SenseDistDot=off  SenseIncDot=off  SenseXDDot=off  SenseYDDot=off  SenseZDDot=off  SenseXYZDDot=off  SenseRadDDot=off  SenseAzimDDot=off  SenseDistDDot=off  SenseIncDDot=off
  Transform Sensor1 : sm_lib/Frames and Transforms/Transform Sensor  MeasurementFrame=World  RotationSequence=XYX  SenseAngle=off  SenseAxis=off  SenseQ=on  SenseR=off  SenseRotationSequence=off  SenseOmegaX=on  SenseOmegaY=on  SenseOmegaZ=on  SenseOmega=off  SenseQDot=off  SenseRDot=off  SenseRotationSequenceDot=off  SenseAlphaX=off  SenseAlphaY=off  SenseAlphaZ=off  SenseAlpha=off  SenseQDDot=off  SenseRDDot=off  SenseX=on  SenseY=on  SenseZ=on  SenseXYZ=off  SenseRad=off  SenseAzim=off  SenseDist=off  SenseInc=off  SenseXDot=on  SenseYDot=on  SenseZDot=on  SenseXYZDot=off  SenseRadDot=off  SenseAzimDot=off  SenseDistDot=off  SenseIncDot=off  SenseXDDot=on  SenseYDDot=on  SenseZDDot=on  SenseXYZDDot=off  SenseRadDDot=off  SenseAzimDDot=off  SenseDistDDot=off  SenseIncDDot=off
  F : PMIOPort  Side=Left
  B : PMIOPort  Port=2  Side=Right
  Bus Element Out : Outport  VectorParamsAs1DForOutWhenUnconnected=off  PortName=World  Element=x
  Bus Element Out3 : Outport  VectorParamsAs1DForOutWhenUnconnected=off  PortName=World  Element=y
  Bus Element Out6 : Outport  VectorParamsAs1DForOutWhenUnconnected=off  PortName=World  Element=z
  Bus Element Out1 : Outport  VectorParamsAs1DForOutWhenUnconnected=off  PortName=World  Element=vx
  Bus Element Out4 : Outport  VectorParamsAs1DForOutWhenUnconnected=off  PortName=World  Element=vy
  Bus Element Out7 : Outport  VectorParamsAs1DForOutWhenUnconnected=off  PortName=World  Element=vz
  Bus Element Out2 : Outport  VectorParamsAs1DForOutWhenUnconnected=off  PortName=World  Element=gx
  Bus Element Out5 : Outport  VectorParamsAs1DForOutWhenUnconnected=off  PortName=World  Element=gy
  Bus Element Out8 : Outport  VectorParamsAs1DForOutWhenUnconnected=off  PortName=World  Element=gz
  Bus Element Out9 : Outport  VectorParamsAs1DForOutWhenUnconnected=off  PortName=World  Element=nRoll
  Bus Element Out10 : Outport  VectorParamsAs1DForOutWhenUnconnected=off  PortName=World  Element=nPitch
  Bus Element Out11 : Outport  VectorParamsAs1DForOutWhenUnconnected=off  PortName=World  Element=nYaw
  Bus Element Out12 : Outport  VectorParamsAs1DForOutWhenUnconnected=off  PortName=World  Element=aRoll
  Bus Element Out13 : Outport  VectorParamsAs1DForOutWhenUnconnected=off  PortName=World  Element=aPitch
  Bus Element Out14 : Outport  VectorParamsAs1DForOutWhenUnconnected=off  PortName=World  Element=aYaw
  Out Bus Element : Outport  VectorParamsAs1DForOutWhenUnconnected=off  PortName=World  Element=Q
  wires:
  PS-Simulink Converter1/1 -> Bus Element Out3/1
  PS-Simulink Converter7/1 -> Bus Element Out5/1
  PS-Simulink Converter8/1 -> Bus Element Out8/1
  PS-Simulink Converter9/1 -> Bus Element Out9/1
  PS-Simulink Converter5/1 -> Bus Element Out7/1
  PS-Simulink Converter/1 -> Bus Element Out/1
  PS-Simulink Converter4/1 -> Bus Element Out4/1
  PS-Simulink Converter6/1 -> Bus Element Out2/1
  PS-Simulink Converter2/1 -> Bus Element Out6/1
  PS-Simulink Converter3/1 -> Bus Element Out1/1
  Signal Specification2/1 -> Bus Element Out14/1
  Signal Specification1/1 -> Bus Element Out13/1
  Signal Specification/1 -> Bus Element Out12/1
  PS-Simulink Converter10/1 -> Bus Element Out10/1
  PS-Simulink Converter11/1 -> Bus Element Out11/1
  PS-Simulink Converter12/1 -> Out Bus Element/1
  PS-Simulink Converter13/1 -> R to X-Y-Z Extrinsic/1(R)
  R to X-Y-Z Extrinsic/2(pitch) -> Signal Specification1/1
  R to X-Y-Z Extrinsic/3(roll) -> Signal Specification/1
  R to X-Y-Z Extrinsic/1(yaw) -> Signal Specification2/1
  connections:
  B/RConn1 -- Transform Sensor1/LConn1 -- Rigid Transform/LConn1 -- Transform Sensor/LConn1
  Transform Sensor/RConn1 -- Transform Sensor1/RConn1 -- Rigid Transform/RConn1 -- F/RConn1
  Transform Sensor/RConn2 -- PS-Simulink Converter13/LConn1
  PS-Simulink Converter/LConn1 -- Transform Sensor1/RConn6
  PS-Simulink Converter3/LConn1 -- Transform Sensor1/RConn9
  PS-Simulink Converter6/LConn1 -- Transform Sensor1/RConn12
  PS-Simulink Converter1/LConn1 -- Transform Sensor1/RConn7
  PS-Simulink Converter4/LConn1 -- Transform Sensor1/RConn10
  PS-Simulink Converter2/LConn1 -- Transform Sensor1/RConn8
  PS-Simulink Converter5/LConn1 -- Transform Sensor1/RConn11
  PS-Simulink Converter8/LConn1 -- Transform Sensor1/RConn14
  PS-Simulink Converter7/LConn1 -- Transform Sensor1/RConn13
  PS-Simulink Converter12/LConn1 -- Transform Sensor1/RConn2
  PS-Simulink Converter9/LConn1 -- Transform Sensor1/RConn3
  PS-Simulink Converter10/LConn1 -- Transform Sensor1/RConn4
  PS-Simulink Converter11/LConn1 -- Transform Sensor1/RConn5

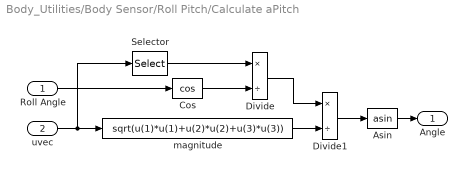
== system Body_Utilities/Body Sensor/Roll Pitch/Calculate aPitch ==
  Roll Angle : Inport
  uvec : Inport  Port=2
  Asin : Trigonometry  Operator=asin
  Cos : Trigonometry  Operator=cos
  Divide : Product  Inputs=*/
  Divide1 : Product  Inputs=*/
  Selector : Selector  InputPortWidth=3  IndexOptions=Index vector (dialog)  Indices=[3]  OutputSizes=1
  magnitude : Fcn  Expr=sqrt(u(1)*u(1)+u(2)*u(2)+u(3)*u(3))
  Angle : Outport  VectorParamsAs1DForOutWhenUnconnected=off
  wires:
  Cos/1 -> Divide/2
  Divide/1 -> Divide1/1
  Asin/1 -> Angle/1
  Roll Angle/1 -> Cos/1
  Selector/1 -> Divide/1
  magnitude/1 -> Divide1/2
  uvec/1 -> Selector/1, magnitude/1
  Divide1/1 -> Asin/1

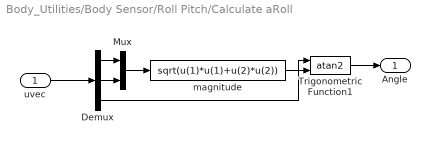
== system Body_Utilities/Body Sensor/Roll Pitch/Calculate aRoll ==
  uvec : Inport
  Demux : Demux  Outputs=3
  Mux : Mux  Inputs=2
  Trigonometric Function1 : Trigonometry  Operator=atan2
  magnitude : Fcn  Expr=sqrt(u(1)*u(1)+u(2)*u(2))
  Angle : Outport  VectorParamsAs1DForOutWhenUnconnected=off
  wires:
  Demux/1 -> Mux/1
  uvec/1 -> Demux/1
  Trigonometric Function1/1 -> Angle/1
  Demux/3 -> Trigonometric Function1/1
  Mux/1 -> magnitude/1
  magnitude/1 -> Trigonometric Function1/2
  Demux/2 -> Mux/2

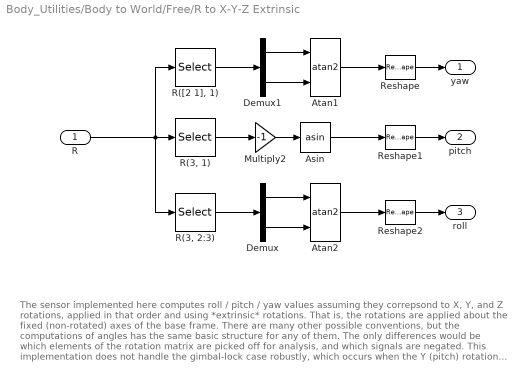
== system Body_Utilities/Body to World/Free/R to X-Y-Z Extrinsic ==
  note: The sensor implemented here computes roll / pitch / yaw values assuming they correpsond to X, Y, and Z rotations, applied in that order and using  *extrinsic* rotations.  That is, the rotations are applied about the fixed (non-rotated) axes of the base frame.   There are many other possible conventions, but the computations of angles has the same basic structure for any of them.  The only differences would be which elements of the rotation matrix are picked off for analysis, and which signals are negated.
      |
      | This implementation does not handle the gimbal-lock case robustly, which occurs when the Y (pitch) rotation is +/-90 degrees.  Handling this case requires a more complex computation,
      | but it can be done with a few more trig blocks and selectors.
  R : Inport
  Asin : Trigonometry  Operator=asin
  Atan1 : Trigonometry  Operator=atan2
  Atan2 : Trigonometry  Operator=atan2
  Demux : Demux  Outputs=2
  Demux1 : Demux  Outputs=2
  Multiply2 : Gain  Gain=-1
  "R(3, 1)" : Selector  NumberOfDimensions=2  InputPortWidth=3  IndexOptions=Index vector (dialog),Index vector (dialog)  Indices=3,1  OutputSizes=1,1
  "R(3, 2:3)" : Selector  NumberOfDimensions=2  InputPortWidth=3  IndexOptions=Index vector (dialog),Index vector (dialog)  Indices=3,[2 3]  OutputSizes=1,1
  "R([2 1], 1)" : Selector  NumberOfDimensions=2  InputPortWidth=3  IndexOptions=Index vector (dialog),Index vector (dialog)  Indices=[2 1],1  OutputSizes=1,1
  Reshape : Reshape
  Reshape1 : Reshape
  Reshape2 : Reshape  OutputDimensionality=Customize  OutputDimensions=1
  yaw : Outport  VectorParamsAs1DForOutWhenUnconnected=off
  pitch : Outport  Port=2  VectorParamsAs1DForOutWhenUnconnected=off
  roll : Outport  Port=3  VectorParamsAs1DForOutWhenUnconnected=off
  wires:
  Reshape2/1 -> roll/1
  Reshape1/1 -> pitch/1
  Reshape/1 -> yaw/1
  Atan1/1 -> Reshape/1
  "R(3, 2:3)"/1 -> Demux/1
  Multiply2/1 -> Asin/1
  "R([2 1], 1)"/1 -> Demux1/1
  Demux1/1 -> Atan1/1
  R/1 -> "R([2 1], 1)"/1, "R(3, 2:3)"/1, "R(3, 1)"/1
  Asin/1 -> Reshape1/1
  "R(3, 1)"/1 -> Multiply2/1
  Atan2/1 -> Reshape2/1
  Demux/2 -> Atan2/2
  Demux1/2 -> Atan1/2
  Demux/1 -> Atan2/1

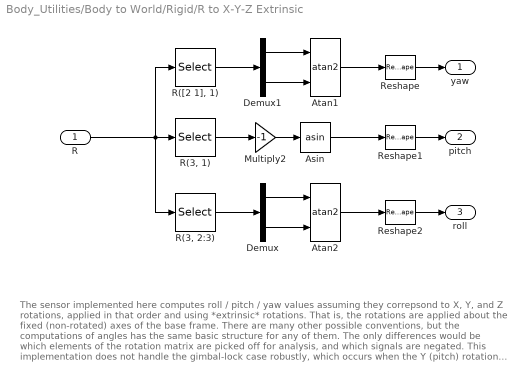
== system Body_Utilities/Body to World/Rigid/R to X-Y-Z Extrinsic ==
  note: The sensor implemented here computes roll / pitch / yaw values assuming they correpsond to X, Y, and Z rotations, applied in that order and using  *extrinsic* rotations.  That is, the rotations are applied about the fixed (non-rotated) axes of the base frame.   There are many other possible conventions, but the computations of angles has the same basic structure for any of them.  The only differences would be which elements of the rotation matrix are picked off for analysis, and which signals are negated.
      |
      | This implementation does not handle the gimbal-lock case robustly, which occurs when the Y (pitch) rotation is +/-90 degrees.  Handling this case requires a more complex computation,
      | but it can be done with a few more trig blocks and selectors.
  R : Inport
  Asin : Trigonometry  Operator=asin
  Atan1 : Trigonometry  Operator=atan2
  Atan2 : Trigonometry  Operator=atan2
  Demux : Demux  Outputs=2
  Demux1 : Demux  Outputs=2
  Multiply2 : Gain  Gain=-1
  "R(3, 1)" : Selector  NumberOfDimensions=2  InputPortWidth=3  IndexOptions=Index vector (dialog),Index vector (dialog)  Indices=3,1  OutputSizes=1,1
  "R(3, 2:3)" : Selector  NumberOfDimensions=2  InputPortWidth=3  IndexOptions=Index vector (dialog),Index vector (dialog)  Indices=3,[2 3]  OutputSizes=1,1
  "R([2 1], 1)" : Selector  NumberOfDimensions=2  InputPortWidth=3  IndexOptions=Index vector (dialog),Index vector (dialog)  Indices=[2 1],1  OutputSizes=1,1
  Reshape : Reshape
  Reshape1 : Reshape
  Reshape2 : Reshape  OutputDimensionality=Customize  OutputDimensions=1
  yaw : Outport  VectorParamsAs1DForOutWhenUnconnected=off
  pitch : Outport  Port=2  VectorParamsAs1DForOutWhenUnconnected=off
  roll : Outport  Port=3  VectorParamsAs1DForOutWhenUnconnected=off
  wires:
  Demux/1 -> Atan2/1
  Demux1/2 -> Atan1/2
  Demux/2 -> Atan2/2
  Atan2/1 -> Reshape2/1
  "R(3, 1)"/1 -> Multiply2/1
  Asin/1 -> Reshape1/1
  R/1 -> "R(3, 1)"/1, "R(3, 2:3)"/1, "R([2 1], 1)"/1
  Demux1/1 -> Atan1/1
  "R([2 1], 1)"/1 -> Demux1/1
  Multiply2/1 -> Asin/1
  "R(3, 2:3)"/1 -> Demux/1
  Atan1/1 -> Reshape/1
  Reshape/1 -> yaw/1
  Reshape1/1 -> pitch/1
  Reshape2/1 -> roll/1
